simulink model "exo_rehab_system"  (R2024b)
settings: Solver=ode4  StartTime=0.0  StopTime=20.0  FixedStep=0.001  RelTol=1e-3
PreLoadFcn:
  | cd('E:\college\ICT\1\exo_project'); addpath(genpath(pwd));
InitFcn:
  | cd('E:\college\ICT\1\exo_project');addpath(genpath(pwd));load('exo_workspace.mat', 'p', 'ctrl', 'fis_cg_data');
undefined symbols (not defined in the file or in its folder): ctrl, p
libraries: slpidlib x1
settings Model: Creator=33242  LastModifiedBy=33242

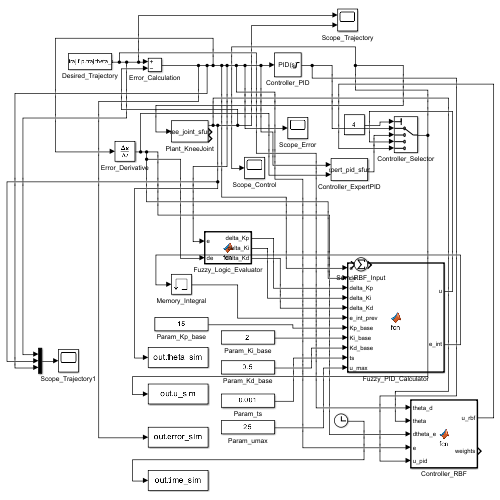
[thumbnail: Simulink's stored preview of the top-level diagram]
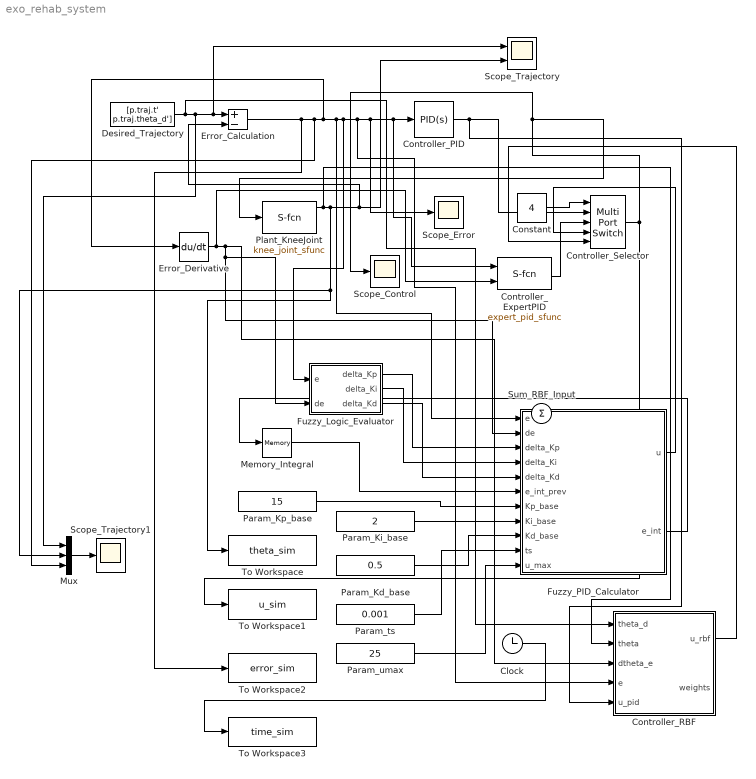
== system exo_rehab_system ==
  Clock : Clock
  Constant : Constant  Value=4
  Controller_ExpertPID : M-S-Function  FunctionName=expert_pid_sfunc  Parameters=ctrl.expert.Kp, ctrl.expert.Ki, ctrl.expert.Kd, ctrl.expert.M1, ctrl.expert.M2, ctrl.expert.eps, ctrl.expert.k1, ctrl.expert.k2, ctrl.expert.umax, p.dt
  Controller_PID : slpidlib/PID Controller  Controller=PID  Form=Parallel  TimeDomain=Continuous-time  UseExternalTs=off  SampleTime=-1  IntegratorMethod=Forward Euler  FilterMethod=Forward Euler  ControllerParametersSource=internal  P=ctrl.pid.Kp  I=ctrl.pid.Ki  UseKiTs=off  D=ctrl.pid.Kd  UseExternalDerivativeSource=off  N=100  UseFilter=on  TunerSelectOption=Transfer Function Based (PID Tuner App)  InitialConditionSource=internal  InitialConditionForIntegrator=0  InitialConditionForFilter=0  DifferentiatorICPrevScaledInput=0  ExternalReset=none  TrackingMode=off  Kt=1  LimitOutput=on  SatLimitsSource=internal  UpperSaturationLimit=p.u_max  LowerSaturationLimit=-p.u_max  LinearizeAsGain=on  AntiWindupMode=none  Kb=1  LimitIntegrator=off  UpperIntegratorSaturationLimit=inf  LowerIntegratorSaturationLimit=-inf  POutMin=[]  POutMax=[]  IOutMin=[]  IOutMax=[]  DOutMin=[]  DOutMax=[]  NOutMin=[]  NOutMax=[]  SumOutMin=[]  SumOutMax=[]  SaturationOutMin=[]  SaturationOutMax=[]  PParamMin=[]  PParamMax=[]  IParamMin=[]  IParamMax=[]  DParamMin=[]  DParamMax=[]  NParamMin=[]  NParamMax=[]  KbParamMin=[]  KbParamMax=[]  KtParamMin=[]  KtParamMax=[]  KbOutMin=[]  KbOutMax=[]  KtOutMin=[]  KtOutMax=[]  IntegratorOutMin=[]  IntegratorOutMax=[]  FilterOutMin=[]  FilterOutMax=[]  SumI1OutMin=[]  SumI1OutMax=[]  SumI2OutMin=[]  SumI2OutMax=[]  SumI3OutMin=[]  SumI3OutMax=[]  SumI4OutMin=[]  SumI4OutMax=[]  SumDOutMin=[]  SumDOutMax=[]  DifferentiatorOutMin=[]  DifferentiatorOutMax=[]  FilterDiffOutCoefMin=[]  FilterDiffOutCoefMax=[]  ReciprocalOutMin=[]  ReciprocalOutMax=[]  SumDenOutMin=[]  SumDenOutMax=[]  SumNumOutMin=[]  SumNumOutMax=[]  DivideOutMin=[]  DivideOutMax=[]  UdiffTsProdOutMin=[]  UdiffTsProdOutMax=[]  NTsProdOutMin=[]  NTsProdOutMax=[]  UintegralTsProdOutMin=[]  UintegralTsProdOutMax=[]  UngainTsProdOutMin=[]  UngainTsProdOutMax=[]  ClampingZeroOutDataTypeStr=Inherit: Inherit via back propagation  ClampingZeroOutMin=[]  ClampingZeroOutMax=[]  FilterDenConstantOutDataTypeStr=Inherit: Inherit via back propagation  FilterDenConstantOutMin=[]  FilterDenConstantOutMax=[]  PCopyOutDataTypeStr=Inherit: Inherit via back propagation  PCopyOutMin=[]  PCopyOutMax=[]  NCopyOutDataTypeStr=Inherit: Inherit via back propagation  NCopyOutMin=[]  NCopyOutMax=[]  IntegratorContinuousStateAttributes=''  IntegratorStateMustResolveToSignalObject=off  IntegratorRTWStateStorageClass=Auto  FilterContinuousStateAttributes=''  FilterStateMustResolveToSignalObject=off  FilterRTWStateStorageClass=Auto  ParallelPVariant=InternalParameters  IdealPVariant=Disabled  IVariant=InternalParameters  DVariant=InternalParameters  IntegratorVariant=Continuous  SatVariant=Enabled  AWVariant=Passthrough  PCopyVariant=Disabled  TRVariant=Disabled  FdbkBlocksVariant=Forward  IdealPFdbkVariant=Disabled  SatFdbkVariant=Disabled  DerivativeFilterVariant=ContFilter  NVariant=InternalParameters  NCopyVariant=Disabled  FilterICVariant=InternalICsFilter  IntegratorICVariant=InternalICs  ExternalResetVariant=Disabled  TRSumVariant=Passthrough  SumFdbkVariant=Disabled  SumVariant=Sum_PID  TsampFilterVariant=InternalTs  TsampNgainVariant=Passthrough  TsampIntegralVariant=Disabled_SignalSpec  ExternalSaturationOutDataTypeStr=Inherit: Same as second input  DerivativeSourceVariant=ErrorSignal  PreIntVariant=InternalPreInt
  Controller_RBF : MATLAB Function  TreatAsAtomicUnit=on  SystemSampleTime=0.001
  Controller_Selector : MultiPortSwitch  Inputs=4  SaturateOnIntegerOverflow=off  InputSameDT=off
  Desired_Trajectory : FromWorkspace  VariableName=[p.traj.t' p.traj.theta_d']
  Error_Calculation : Sum  Inputs=+-
  Error_Derivative : Derivative
  Fuzzy_Logic_Evaluator : MATLAB Function  TreatAsAtomicUnit=on
  Fuzzy_PID_Calculator : MATLAB Function  TreatAsAtomicUnit=on
  Memory_Integral : Memory
  Mux : Mux  Inputs=3
  Param_Kd_base : Constant  Value=0.5
  Param_Ki_base : Constant  Value=2
  Param_Kp_base : Constant  Value=15
  Param_ts : Constant  Value=0.001
  Param_umax : Constant  Value=25
  Plant_KneeJoint : M-S-Function  FunctionName=knee_joint_sfunc  Parameters=p.J, p.B, p.K, p.Fc, p.Fv, p.Fs, p.vs, p.sim_time, p.fatigue_tau, p.tau_patient_max, p.spasm_amp, p.spasm_duration, p.spasm_interval, p.noise_angle, p.noise_velocity, p.J_perturb_amp, p.J_perturb_freq
  Scope_Control : Scope
  Scope_Error : Scope
  Scope_Trajectory : Scope  NumInputPorts=2
  Scope_Trajectory1 : Scope
  Sum_RBF_Input : Sum  Inputs=+
  To Workspace : ToWorkspace  VariableName=theta_sim  SampleTime=-1
  To Workspace1 : ToWorkspace  VariableName=u_sim  SampleTime=-1
  To Workspace2 : ToWorkspace  VariableName=error_sim  SampleTime=-1
  To Workspace3 : ToWorkspace  VariableName=time_sim  SampleTime=-1
  wires:
  Desired_Trajectory/1 -> Controller_RBF/1(theta_d), Mux/1, Error_Calculation/1, Scope_Trajectory/1
  Plant_KneeJoint/1 -> Controller_RBF/2(theta), Mux/2, To Workspace/1, Scope_Trajectory/2, Error_Calculation/2
  Controller_PID/1 -> Controller_RBF/5(u_pid), Controller_Selector/2
  Controller_Selector/1 -> Scope_Control/1, Plant_KneeJoint/1, To Workspace1/1
  Error_Derivative/1 -> Controller_RBF/3(dtheta_e), Fuzzy_Logic_Evaluator/2(de), Fuzzy_PID_Calculator/2(de), Controller_ExpertPID/2
  Controller_ExpertPID/1 -> Controller_Selector/3
  Constant/1 -> Controller_Selector/1
  Clock/1 -> To Workspace3/1
  Mux/1 -> Scope_Trajectory1/1
  Error_Calculation/1 -> To Workspace2/1, Mux/3, Fuzzy_Logic_Evaluator/1(e), Controller_RBF/4(e), Scope_Error/1, Controller_ExpertPID/1, Controller_PID/1, Fuzzy_PID_Calculator/1(e), Error_Derivative/1
  Fuzzy_Logic_Evaluator/1(delta_Kp) -> Fuzzy_PID_Calculator/3(delta_Kp)
  Fuzzy_Logic_Evaluator/2(delta_Ki) -> Fuzzy_PID_Calculator/4(delta_Ki)
  Fuzzy_Logic_Evaluator/3(delta_Kd) -> Fuzzy_PID_Calculator/5(delta_Kd)
  Fuzzy_PID_Calculator/2(e_int) -> Memory_Integral/1
  Memory_Integral/1 -> Fuzzy_PID_Calculator/6(e_int_prev)
  Param_Kp_base/1 -> Fuzzy_PID_Calculator/7(Kp_base)
  Param_Ki_base/1 -> Fuzzy_PID_Calculator/8(Ki_base)
  Param_Kd_base/1 -> Fuzzy_PID_Calculator/9(Kd_base)
  Param_ts/1 -> Fuzzy_PID_Calculator/10(ts)
  Param_umax/1 -> Fuzzy_PID_Calculator/11(u_max)
  Fuzzy_PID_Calculator/1(u) -> Controller_Selector/4
  Controller_RBF/1(u_rbf) -> Controller_Selector/5

== matlab function exo_rehab_system/Fuzzy_Logic_Evaluator ==
  data: e input; delta_Kp output; de input; delta_Ki output; delta_Kd output
function [delta_Kp, delta_Ki, delta_Kd] = fcn(e, de)
%#codegen
% Fuzzy Logic Evaluator - Code Generation Compatible
% Complete fuzzy inference hard-coded (no external FIS file)

%% Input Normalization
% e: error in [-pi/2, pi/2] -> normalize to [-1, 1]
% de: error rate in [-pi/4, pi/4] -> normalize to [-1, 1]

e_max = 1.5708;   % pi/2
de_max = 0.7854;  % pi/4

e_norm = max(-1, min(1, e / e_max));
de_norm = max(-1, min(1, de / de_max));

%% Fuzzy Membership Functions
% 7 fuzzy levels: NB, NM, NS, ZE, PS, PM, PB
% Centers: -1.0, -0.67, -0.33, 0.0, 0.33, 0.67, 1.0

% Membership function calculation (Triangular)
e_mf = calculate_membership(e_norm);
de_mf = calculate_membership(de_norm);

%% Fuzzy Rule Base (49 rules)
% Output levels (5): NB=1, NS=2, ZE=3, PS=4, PB=5

% Rule table for delta_Kp (7x7)
dKp_rules = int8([
    5, 5, 4, 4, 4, 5, 5;
    5, 4, 4, 3, 4, 4, 5;
    4, 4, 3, 3, 3, 4, 4;
    3, 3, 3, 3, 3, 3, 3;
    4, 4, 3, 3, 3, 4, 4;
    5, 4, 4, 3, 4, 4, 5;
    5, 5, 4, 4, 4, 5, 5
]);

% Rule table for delta_Ki (7x7)
dKi_rules = int8([
    1, 1, 1, 1, 1, 1, 1;
    1, 1, 2, 2, 2, 1, 1;
    2, 2, 3, 3, 3, 2, 2;
    3, 4, 4, 5, 4, 4, 3;
    2, 2, 3, 3, 3, 2, 2;
    1, 1, 2, 2, 2, 1, 1;
    1, 1, 1, 1, 1, 1, 1
]);

% Rule table for delta_Kd (7x7)
dKd_rules = int8([
    5, 4, 3, 3, 3, 4, 5;
    4, 4, 3, 2, 3, 4, 4;
    3, 3, 3, 2, 3, 3, 3;
    2, 2, 2, 2, 2, 2, 2;
    3, 3, 3, 2, 3, 3, 3;
    4, 4, 3, 2, 3, 4, 4;
    5, 4, 3, 3, 3, 4, 5
]);

%% Fuzzy Inference (Mamdani method)
dKp_out = zeros(5, 1);
dKi_out = zeros(5, 1);
dKd_out = zeros(5, 1);

% Apply all 49 rules
for i = 1:7
    for j = 1:7
        % Calculate firing strength (min operator)
        strength = min(e_mf(i), de_mf(j));
        
        % Aggregate outputs (max operator)
        idx_Kp = dKp_rules(i, j);
        idx_Ki = dKi_rules(i, j);
        idx_Kd = dKd_rules(i, j);
        
        dKp_out(idx_Kp) = max(dKp_out(idx_Kp), strength);
        dKi_out(idx_Ki) = max(dKi_out(idx_Ki), strength);
        dKd_out(idx_Kd) = max(dKd_out(idx_Kd), strength);
    end
end

%% Defuzzification (Centroid method)
% Output universe of discourse
Kp_centers = [-10.0, -5.0, 0.0, 5.0, 10.0];
Ki_centers = [-0.5, -0.25, 0.0, 0.25, 0.5];
Kd_centers = [-1.0, -0.5, 0.0, 0.5, 1.0];

% Centroid calculation
delta_Kp = centroid(Kp_centers, dKp_out);
delta_Ki = centroid(Ki_centers, dKi_out);
delta_Kd = centroid(Kd_centers, dKd_out);

end

%% Local Functions

function mf = calculate_membership(x)
% Calculate membership degrees for 7 fuzzy sets
% x: normalized input in [-1, 1]

mf = zeros(7, 1);
centers = [-1.0, -0.67, -0.33, 0.0, 0.33, 0.67, 1.0];
width = 0.33;

for i = 1:7
    if i == 1
        % Leftmost (trapezoidal)
        if x <= centers(1)
            mf(i) = 1.0;
        elseif x <= centers(2)
            mf(i) = (centers(2) - x) / width;
        else
            mf(i) = 0.0;
        end
    elseif i == 7
        % Rightmost (trapezoidal)
        if x >= centers(7)
            mf(i) = 1.0;
        elseif x >= centers(6)
            mf(i) = (x - centers(6)) / width;
        else
            mf(i) = 0.0;
        end
    else
        % Middle (triangular)
        dist = abs(x - centers(i));
        if dist <= width
            mf(i) = 1.0 - dist / width;
        else
            mf(i) = 0.0;
        end
    end
end

end

function result = centroid(centers, membership)
% Centroid defuzzification
% centers: output universe centers
% membership: membership degrees

numerator = 0.0;
denominator = 0.0;

for i = 1:length(centers)
    numerator = numerator + centers(i) * membership(i);
    denominator = denominator + membership(i);
end

% Avoid division by zero
if denominator < 0.001
    result = 0.0;
else
    result = numerator / denominator;
end

end

== matlab function exo_rehab_system/Fuzzy_PID_Calculator ==
  data: e input; u output; de input; delta_Kp input; delta_Ki input; delta_Kd input; e_int_prev input; Kp_base input; Ki_base input; Kd_base input; ts input; u_max input; e_int output
function [u, e_int] = fcn(e, de, delta_Kp, delta_Ki, delta_Kd, e_int_prev, Kp_base, Ki_base, Kd_base, ts, u_max)
%#codegen
% Fuzzy PID Calculator - No Chinese characters

% Compute adaptive PID parameters
Kp = max(0.1, Kp_base + delta_Kp);
Ki = max(0.0, Ki_base + delta_Ki);
Kd = max(0.0, Kd_base + delta_Kd);

% Compute error integral
e_int = e_int_prev + e * ts;

% Anti-windup
I_max = u_max / max(Ki, 0.01);
e_int = max(-I_max, min(I_max, e_int));

% PID control law
u = Kp * e + Ki * e_int + Kd * de;

% Output saturation
u = max(-u_max, min(u_max, u));

end

== matlab function exo_rehab_system/Controller_RBF ==
  data: theta_d input; u_rbf output; theta input; dtheta_e input; e input; u_pid input; weights output
function [u_rbf, weights] = fcn(theta_d, theta, dtheta_e, e, u_pid)
%#codegen
% Simplified RBF Adaptive Controller
% Inputs: theta_d, theta, dtheta_e, e (error), u_pid (baseline)
% Outputs: u_rbf (compensation), weights (for monitoring)

%% RBF Network Parameters (hard-coded for code generation)
n_hidden = 11;
eta = 0.05;
lambda = 0.99;
u_max = 25.0;

%% Persistent variables (weights and centers)
persistent w centers sigma

if isempty(w)
    % Initialize weights
    w = 0.01 * randn(n_hidden, 1);
    
    % Initialize RBF centers (uniform distribution)
    centers = zeros(n_hidden, 3);
    theta_range = linspace(0, pi/2, 4);
    dtheta_range = linspace(-pi/4, pi/4, 3);
    
    idx = 1;
    for i = 1:4
        for j = 1:3
            if idx > n_hidden
                break;
            end
            centers(idx, 1) = theta_range(i);
            centers(idx, 2) = theta_range(i);
            centers(idx, 3) = dtheta_range(j);
            idx = idx + 1;
        end
    end
    
    % Initialize sigma
    sigma = 0.3 * ones(n_hidden, 1);
end

%% Construct input vector
x = [theta_d; theta; dtheta_e];

%% Calculate RBF activations
phi = zeros(n_hidden, 1);
for j = 1:n_hidden
    diff = x - centers(j, :)';
    phi(j) = exp(-sum(diff.^2) / (2 * sigma(j)^2));
end

%% RBF output (uncertainty compensation)
f_hat = w' * phi;

%% Total control (PID + RBF compensation)
u_rbf = u_pid + 0.3 * f_hat;  % Scale down compensation

%% Output saturation
u_rbf = max(-u_max, min(u_max, u_rbf));

%% Weight update (gradient descent + decay)
ts = 0.001;  % Sample time
delta_w = ts * (eta * e * phi - lambda * w);
w = w + delta_w;

%% Weight limiting (prevent explosion)
w_max = 30.0;
w = max(-w_max, min(w_max, w));

%% Output weights for monitoring
weights = w;

end
